simulink model "pv_model_F9_module_mismatch"  (R2025b)
settings: Solver=FixedStepDiscrete  StartTime=0.0  StopTime=86400  FixedStep=1  RelTol=1e-3  AbsTol=1e-6
PreLoadFcn:
  | power_PVarray_250kW_param;
InitFcn:
  | power_PVarray_250kW_param;
undefined symbols (not defined in the file): Rload_day, Ts_Control, Ts_Power, Vnom_dc
libraries: spsPVArrayLib x15, spsCurrentMeasurementLib x7, spsPVarrayModel x2, spsMeanLib x2, spsSeriesRLCBranchLib x1, spsVoltageMeasurementLib x1, spspowerguiLib x1
Description:
  | Copyright 2008-2017 The MathWorks, Inc.
settings Model: Creator=MathWorks  LastModifiedBy=edgar
settings DataIOCC: LimitDataPoints=on  SaveFormat=Array  SignalLoggingSaveFormat=ModelDataLogs  DSMLogging=off  ReturnWorkspaceOutputs=off
settings OptimizationCC: ExpressionDepthLimit=2147483647.0  LifeSpan=inf
settings DebuggingCC: AlgebraicLoopMsg=none  UnderspecifiedInitializationDetection=Classic  MergeDetectMultiDrivingBlocksExec=none  SolverPrmCheckMsg=warning  FcnCallInpInsideContextMsg=warning  UnconnectedInputMsg=warning  UnconnectedOutputMsg=warning  UnconnectedLineMsg=warning  StateNameClashWarn=warning  SFUnexpectedBacktrackingDiag=warning  SFNoUnconditionalDefaultTransitionDiag=warning  SFExecutionAtInitializationDiag=none  ArithmeticOperatorsInVariantConditions=warning
settings HardwareCC: ProdBitPerPointer=32.0  ProdBitPerSizeT=32.0  ProdBitPerPtrDiffT=32.0  ProdLargestAtomicFloat=None  ProdIntDivRoundTo=Undefined  ProdEndianess=Unspecified  ProdWordSize=32.0  ProdHWDeviceType=32-bit Generic
settings ModelReferenceCC: EnableRefExpFcnMdlSchedulingChecks=on  PropagateSignalLabelsOutOfModel=off
settings SFSimCC: SimUseLocalCustomCode=off  CustomCodeUndefinedFunction=UseInterfaceOnly
settings RTWCC: RTWUseLocalCustomCode=off  GPUComputeCapability=3.5
settings CodeAppCC: StateflowObjectComments=on
settings GRTTargetCC: TargetLangStandard=C89/C90 (ANSI)  CombineOutputUpdateFcns=off  GRTInterface=on
settings ConfigComp: CovMetricSettings=dw  CovSaveCumulativeToWorkspaceVar=on  CovSaveSingleToWorkspaceVar=on  CovExternalEMLEnable=off  CovSFcnEnable=off
settings SimscapeCC: SimscapeNormalizeSystem=off

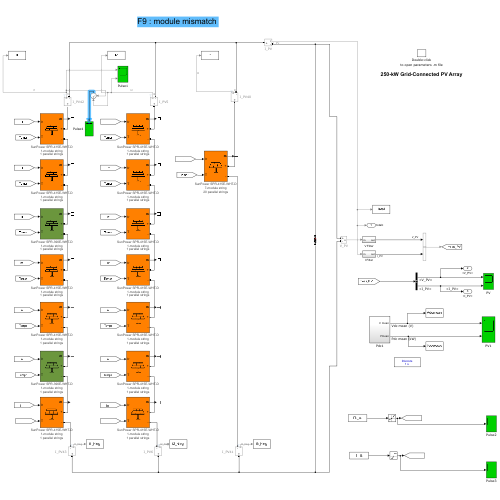
[thumbnail: Simulink's stored preview of the top-level diagram]
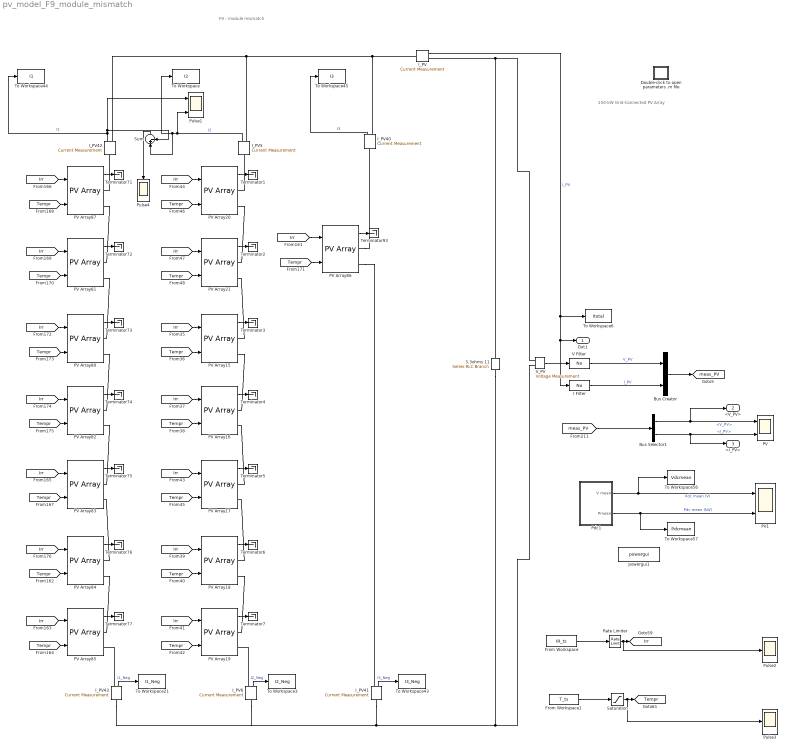
== system pv_model_F9_module_mismatch ==
  note: 250-kW Grid-Connected PV Array
  note: F9 : module mismatch
  3.3ohms 11 : spsSeriesRLCBranchLib/Series RLC Branch  LConnTagsString=__new0  RConnTagsString=__new0  BranchType=R  Resistance=Rload_day  Inductance=[]  SetiL0=off  InitialCurrent=0  Capacitance=[]  Setx0=off  InitialVoltage=0  Measurements=None
  Bus Creator : BusCreator  Inputs=2
  Bus Selector1 : BusSelector  OutputSignals=V_PV,I_PV
  Double-click to open parameters .m file : Subsystem
      settings: OpenFcn=open('power_PVarray_250kW_param.m')
  From Workspace : FromWorkspace  VariableName=IR_ts  SampleTime=1
  From Workspace1 : FromWorkspace  VariableName=T_ts  SampleTime=1
  I Filter : spsPVarrayModel/No  SystemSampleTime=-1  VariantControl=Variant1  VariantActivationTime=update diagram  EmptyChoice=off  PassThrough=off  PassThroughVariantControl=(default)  EmptyChoiceVariantControl=(default)  AllowFlexibleInterface=on  Latency=0  AutoFrameSizeCalculation=off
  I_PV{,5..6,40..43} (7 alike) : spsCurrentMeasurementLib/Current Measurement  PhasorSimulation=off  OutputType=Complex  PSBequivalent=0
  PV : Scope  NumInputPorts=2
      settings: TimeSpan=1.5  ActiveDisplayYMinimum=-71.710124808649638  ActiveDisplayYMaximum=645.39088592996507  DataLoggingDecimation=10  DataLoggingSaveFormat=Array
  PV Array{15..21,81..83,85,87} (12 alike) : spsPVArrayLib/PV Array  Npar=1  Nser=1  PlotType=array @ 1000 W/m2 & specified temperatures  S_vec="[ 1000  500  100 ]"  Temp_C_vec="[ 45 25  ]"  ModuleName=SunPower SPR-415E-WHT-D  PlotWhenSelected=off  Pm=414.801  Ncell=128  Voc=85.3  Isc=6.09  Vm=72.9  Im=5.69  beta_Voc_pc=-0.229  alpha_Isc_pc=0.030706  beta_Voc=-0.19534  alpha_Isc=0.00187  IL=6.0978  I0=7.1698e-13  nI=0.87223  Rsh=419.7781  Rs=0.53711  RobustModel=off  RobustCellTemperature=313.3991  BAL=off  Tc=1e-6  Tfilter=5e-5
      settings: AttributesFormatString=|
      | %<ModuleName>
      | %<Nser>-module string
      | %<Npar> parallel strings
  PV Array80 : spsPVArrayLib/PV Array  Npar=1  Nser=1  PlotType=array @ 1000 W/m2 & specified temperatures  S_vec="[ 1000  500  100 ]"  Temp_C_vec="[ 45 25  ]"  ModuleName=SunPower SPR-390E-WHT-D  PlotWhenSelected=off  Pm=390.015  Ncell=128  Voc=85.3  Isc=5.72  Vm=72.9  Im=5.35  beta_Voc_pc=-0.229  alpha_Isc_pc=0.030699  beta_Voc=-0.19534  alpha_Isc=0.001756  IL=5.727  I0=6.7383e-13  nI=0.87221  Rsh=464.6101  Rs=0.57182  RobustModel=off  RobustCellTemperature=313.3991  BAL=off  Tc=1e-6  Tfilter=5e-5
      settings: AttributesFormatString=|
      | %<ModuleName>
      | %<Nser>-module string
      | %<Npar> parallel strings
  PV Array84 : spsPVArrayLib/PV Array  Npar=1  Nser=1  PlotType=array @ 1000 W/m2 & specified temperatures  S_vec="[ 1000  500  100 ]"  Temp_C_vec="[ 45 25  ]"  ModuleName=SunPower SPR-390E-WHT-D  PlotWhenSelected=off  Pm=390.015  Ncell=128  Voc=85.3  Isc=5.72  Vm=72.9  Im=5.35  beta_Voc_pc=-0.229  alpha_Isc_pc=0.030699  beta_Voc=-0.19534  alpha_Isc=0.001756  IL=5.727  I0=6.7383e-13  nI=0.87221  Rsh=464.6101  Rs=0.57182  RobustModel=off  RobustCellTemperature=313.3991  BAL=off  Tc=1e-6  Tfilter=5e-5
      settings: AttributesFormatString=|
      | %<ModuleName>
      | %<Nser>-module string
      | %<Npar> parallel strings
  PV Array86 : spsPVArrayLib/PV Array  Npar=20  Nser=7  PlotType=array @ 1000 W/m2 & specified temperatures  S_vec="[ 1000  500  100 ]"  Temp_C_vec="[ 45 25  ]"  ModuleName=SunPower SPR-415E-WHT-D  PlotWhenSelected=off  Pm=414.801  Ncell=128  Voc=85.3  Isc=6.09  Vm=72.9  Im=5.69  beta_Voc_pc=-0.229  alpha_Isc_pc=0.030706  beta_Voc=-0.19534  alpha_Isc=0.00187  IL=6.0978  I0=7.1698e-13  nI=0.87223  Rsh=419.7781  Rs=0.53711  RobustModel=off  RobustCellTemperature=313.3991  BAL=off  Tc=1e-6  Tfilter=5e-5
      settings: AttributesFormatString=|
      | %<ModuleName>
      | %<Nser>-module string
      | %<Npar> parallel strings
  PV1 : Scope  NumInputPorts=2
      settings: TimeSpan=1.5  ActiveDisplayYMinimum=208.04916  ActiveDisplayYMaximum=527.55759  DataLoggingDecimation=10  DataLoggingVariableName=ScopeData15  DataLoggingSaveFormat=Array
  Pdc1 : Subsystem
  Pulse1 : Scope  NumInputPorts=2
      settings: TimeSpan=1.5  ActiveDisplayYMinimum=-118.4528917980434  ActiveDisplayYMaximum=1066.0760261823907  DataLoggingDecimation=10  DataLoggingSaveFormat=Array
  Pulse2 : Scope
      settings: TimeSpan=1.5  ActiveDisplayYMinimum=-118.4528917980434  ActiveDisplayYMaximum=1066.0760261823907  DataLoggingDecimation=10  DataLoggingVariableName=ScopeData12  DataLoggingSaveFormat=Array
  Pulse3 : Scope
      settings: TimeSpan=1.5  ActiveDisplayYMinimum=14.376202367904177  ActiveDisplayYMaximum=30.614178688862403  DataLoggingDecimation=10  DataLoggingVariableName=ScopeData13  DataLoggingSaveFormat=Array
  Pulse4 : Scope
      settings: TimeSpan=1.5  ActiveDisplayYMinimum=-118.4528917980434  ActiveDisplayYMaximum=1066.0760261823907  DataLoggingDecimation=10  DataLoggingVariableName=ScopeData2  DataLoggingSaveFormat=Array
  Rate Limiter : RateLimiter  RisingSlewLimit=6000  FallingSlewLimit=-6000  SampleTimeMode=inherited  InitialCondition=1000
  Saturation : Saturate  UpperLimit=55  LowerLimit=5
  Sum : Sum  Inputs=|+-
  Terminator{1..7,71..77,93} (15 alike) : Terminator
  To Workspace : ToWorkspace  VariableName=I2  SampleTime=-1
      settings: Save2DSignal=2-D array (concatenate along first dimension)
  To Workspace21 : ToWorkspace  VariableName=I1_Neg  SampleTime=-1
      settings: Save2DSignal=2-D array (concatenate along first dimension)
  To Workspace3 : ToWorkspace  VariableName=I2_Neg  SampleTime=-1
      settings: Save2DSignal=2-D array (concatenate along first dimension)
  To Workspace43 : ToWorkspace  VariableName=I3_Neg  SampleTime=-1
      settings: Save2DSignal=2-D array (concatenate along first dimension)
  To Workspace44 : ToWorkspace  VariableName=I1  SampleTime=-1
      settings: Save2DSignal=2-D array (concatenate along first dimension)
  To Workspace45 : ToWorkspace  VariableName=I3  SampleTime=-1
      settings: Save2DSignal=2-D array (concatenate along first dimension)
  To Workspace56 : ToWorkspace  VariableName=Vdcmean  SampleTime=-1
      settings: Save2DSignal=2-D array (concatenate along first dimension)
  To Workspace57 : ToWorkspace  VariableName=Pdcmean  SampleTime=-1
      settings: Save2DSignal=2-D array (concatenate along first dimension)
  To Workspace6 : ToWorkspace  VariableName=Itotal  SampleTime=-1
      settings: Save2DSignal=2-D array (concatenate along first dimension)
  V Filter : spsPVarrayModel/No  SystemSampleTime=-1  VariantControl=Variant1  VariantActivationTime=update diagram  EmptyChoice=off  PassThrough=off  PassThroughVariantControl=(default)  EmptyChoiceVariantControl=(default)  AllowFlexibleInterface=on  Latency=0  AutoFrameSizeCalculation=off
  V_PV : spsVoltageMeasurementLib/Voltage Measurement  PhasorSimulation=off  OutputType=Complex  PSBequivalent=0
  powergui1 : spspowerguiLib/powergui  Priority=1  SimulationMode=Discrete  SampleTime=Ts_Power  frequency=60  Iterations=50  frequencyindice=0  Pbase=100e6  ErrMax=1e-4  UnitsV=kV  UnitsW=MW  buscounter=0  FunctionMessages=off  echomessages=off  EnableUseOfTLC=off  CurrentSourceSwitches=off  DisableSnubberDevices=off  DisableRonSwitches=off  DisableVfSwitches=off  DisplayEquations=off  AutomaticDiscreteSolvers=off  SolverType=Tustin  Interpol=off  ExternalGateDelay=off  methode=off  Ts=0  x0status=blocks  SPID=off  SwTol=0  HookPort=off  NonlinearTolerance=1e-4  nMaxIteration=100  ContinueOnMaxIteration=off  RestoreLinks=warning  ResistiveCurrentMeasurement=off  Frange=[0:2:500]  Ylog=off  Xlog=on  ShowGrid=off  save=off  variable=ZData  structure=VaIa_Grid  ZoomFFT=off  StartTime=1.4  cycles=3  DisplayStyle=1  fundamental=60  FreqAxis=on  MaxFrequency=5000  frequencyindicesteady=1  RmsSteady=1  display=off
  Out1 : Outport  SignalName=totalc  VectorParamsAs1DForOutWhenUnconnected=off
  <V_PV> : Outport  Port=2
  <I_PV> : Outport  Port=3
  tag scope: Irr=global, Tempr=global, meas_PV=global
  wires:
  [Irr] -> PV Array83/1
  [Tempr] -> PV Array87/2
  [Tempr] -> PV Array81/2
  [Tempr] -> PV Array85/2
  [Irr] -> PV Array86/1
  [Tempr] -> PV Array82/2
  [Irr] -> PV Array80/1
  [Irr] -> PV Array85/1
  [Tempr] -> PV Array80/2
  [Tempr] -> PV Array86/2
  [Irr] -> PV Array81/1
  [Irr] -> PV Array82/1
  [Tempr] -> PV Array84/2
  I_PV40/1 -> To Workspace45/1  "I3"
  [Irr] -> PV Array87/1
  I_PV43/1 -> To Workspace21/1  "I1_Neg"
  [Irr] -> PV Array84/1
  I_PV42/1 -> Pulse1/1, Sum/2, To Workspace44/1  "I1"
  I_PV41/1 -> To Workspace43/1  "I3_Neg"
  [Tempr] -> PV Array83/2
  Pdc1/2(Pmean) -> To Workspace57/1, PV1/2  "Pdc mean (kW)"
  Pdc1/1(V mean) -> To Workspace56/1, PV1/1  "Vdc mean (V)"
  I_PV/1 -> To Workspace6/1, Out1/1, I Filter/1  "I_PV"
  V_PV/1 -> V Filter/1
  V Filter/1 -> Bus Creator/1  "V_PV"
  Bus Creator/1 -> [meas_PV]
  I Filter/1 -> Bus Creator/2  "I_PV"
  Saturation/1 -> Pulse3/1, [Tempr]
  Bus Selector1/2 -> <I_PV>/1, PV/2  "<I_PV>"
  Rate Limiter/1 -> Pulse2/1, [Irr]
  [meas_PV] -> Bus Selector1/1
  Bus Selector1/1 -> PV/1, <V_PV>/1  "<V_PV>"
  From Workspace/1 -> Rate Limiter/1
  From Workspace1/1 -> Saturation/1
  PV Array87/1 -> Terminator71/1
  PV Array81/1 -> Terminator72/1
  PV Array80/1 -> Terminator73/1
  PV Array82/1 -> Terminator74/1
  PV Array83/1 -> Terminator75/1
  PV Array84/1 -> Terminator76/1
  PV Array85/1 -> Terminator77/1
  PV Array86/1 -> Terminator93/1
  [Irr] -> PV Array15/1
  [Tempr] -> PV Array18/2
  [Irr] -> PV Array20/1
  [Tempr] -> PV Array17/2
  [Tempr] -> PV Array19/2
  PV Array17/1 -> Terminator5/1
  PV Array16/1 -> Terminator4/1
  [Irr] -> PV Array19/1
  [Tempr] -> PV Array21/2
  [Tempr] -> PV Array16/2
  PV Array21/1 -> Terminator2/1
  PV Array20/1 -> Terminator1/1
  PV Array15/1 -> Terminator3/1
  PV Array19/1 -> Terminator7/1
  [Irr] -> PV Array16/1
  [Irr] -> PV Array18/1
  [Tempr] -> PV Array15/2
  [Tempr] -> PV Array20/2
  PV Array18/1 -> Terminator6/1
  [Irr] -> PV Array17/1
  I_PV5/1 -> Sum/1, To Workspace/1, Pulse1/2  "I2"
  I_PV6/1 -> To Workspace3/1  "I2_Neg"
  [Irr] -> PV Array21/1
  Sum/1 -> Pulse4/1
  connections:
  3.3ohms 11/RConn1 -- I_PV6/LConn1 -- I_PV43/LConn1 -- I_PV41/LConn1 -- V_PV/LConn2
  PV Array81/RConn2 -- PV Array80/RConn1
  PV Array82/RConn2 -- PV Array83/RConn1
  PV Array86/RConn1 -- I_PV40/LConn1
  PV Array86/RConn2 -- I_PV41/RConn1
  PV Array84/RConn2 -- PV Array85/RConn1
  I_PV43/RConn1 -- PV Array85/RConn2
  PV Array87/RConn1 -- I_PV42/LConn1
  PV Array87/RConn2 -- PV Array81/RConn1
  PV Array84/RConn1 -- PV Array83/RConn2
  PV Array80/RConn2 -- PV Array82/RConn1
  V_PV/LConn1 -- 3.3ohms 11/LConn1 -- I_PV/RConn1
  I_PV40/RConn1 -- I_PV5/RConn1 -- I_PV42/RConn1 -- I_PV/LConn1
  PV Array20/RConn1 -- I_PV5/LConn1
  PV Array18/RConn2 -- PV Array19/RConn1
  I_PV6/RConn1 -- PV Array19/RConn2
  PV Array18/RConn1 -- PV Array17/RConn2
  PV Array17/RConn1 -- PV Array16/RConn2
  PV Array20/RConn2 -- PV Array21/RConn1
  PV Array15/RConn1 -- PV Array21/RConn2
  PV Array15/RConn2 -- PV Array16/RConn1

== system pv_model_F9_module_mismatch/Double-click to open parameters .m file ==

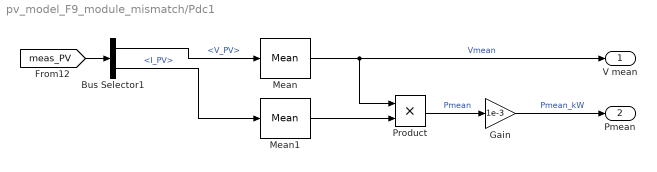
== system pv_model_F9_module_mismatch/Pdc1 ==
  Bus Selector1 : BusSelector  OutputSignals=V_PV,I_PV
  Gain : Gain  Gain=1e-3
  Mean : spsMeanLib/Mean  Freq=Fnom  Vinit=Vnom_dc/2  Ts=Ts_Control
  Mean1 : spsMeanLib/Mean  Freq=Fnom  Vinit=0  Ts=Ts_Control
  Product : Product
  V mean : Outport  VectorParamsAs1DForOutWhenUnconnected=off
  Pmean : Outport  Port=2  VectorParamsAs1DForOutWhenUnconnected=off
  wires:
  Mean/1 -> V mean/1, Product/1  "Vmean"
  Mean1/1 -> Product/2
  Product/1 -> Gain/1  "Pmean"
  Gain/1 -> Pmean/1  "Pmean_kW"
  Bus Selector1/1 -> Mean/1  "<V_PV>"
  Bus Selector1/2 -> Mean1/1  "<I_PV>"
  [meas_PV] -> Bus Selector1/1
